simulink library "Hydraulic_Actuator_Lib"  (R2025a)
settings: Solver=ode45  StartTime=0.0  StopTime=10.0  RelTol=1e-3  EnableMultiTasking=on
undefined symbols (not defined in the file or in its folder): WT_Params
libraries: fl_lib x26, nesl_utility x9, SimscapeFluids_lib x7
Description:
  | Copyright 2009-2025 The MathWorks, Inc. MathWorks, Inc.
settings Model: Creator=smiller  LastModifiedBy=smiller
settings SolverCC: AlgebraicLoopSolver=TrustRegion
settings DataIOCC: LimitDataPoints=on  SaveFormat=Array  SignalLoggingSaveFormat=ModelDataLogs  ReturnWorkspaceOutputs=off
settings OptimizationCC: ReuseModelBlockBuffer=off  ExpressionDepthLimit=2147483647.0  LifeSpan=inf
settings DebuggingCC: UnderspecifiedInitializationDetection=Classic  MergeDetectMultiDrivingBlocksExec=none  SolverPrmCheckMsg=warning  FcnCallInpInsideContextMsg=warning  UnconnectedInputMsg=warning  UnconnectedOutputMsg=warning  UnconnectedLineMsg=warning  AllowSymbolicDim=off  StateNameClashWarn=warning  PregeneratedLibrarySubsystemCodeDiagnostic=none  SFUnexpectedBacktrackingDiag=warning  SFNoUnconditionalDefaultTransitionDiag=warning  SFExecutionAtInitializationDiag=none  ArithmeticOperatorsInVariantConditions=warning
settings HardwareCC: ProdBitPerPointer=32.0  ProdBitPerSizeT=32.0  ProdBitPerPtrDiffT=32.0  ProdLargestAtomicFloat=None  ProdIntDivRoundTo=Undefined  ProdEndianess=Unspecified  ProdWordSize=32.0  ProdHWDeviceType=32-bit Generic
settings ModelReferenceCC: EnableRefExpFcnMdlSchedulingChecks=on  PropagateSignalLabelsOutOfModel=off
settings SFSimCC: SimUseLocalCustomCode=off  CustomCodeUndefinedFunction=UseInterfaceOnly
settings RTWCC: RTWUseLocalCustomCode=off  GPUComputeCapability=3.5  DLArmComputeVersion=19.05
settings CodeAppCC: StateflowObjectComments=on
settings GRTTargetCC: TargetLangStandard=C89/C90 (ANSI)  CombineOutputUpdateFcns=off  GRTInterface=on
settings ConfigComp: CovMetricSettings=dw  CovSaveCumulativeToWorkspaceVar=on  CovSaveSingleToWorkspaceVar=on  CovExternalEMLEnable=off  CovSFcnEnable=off

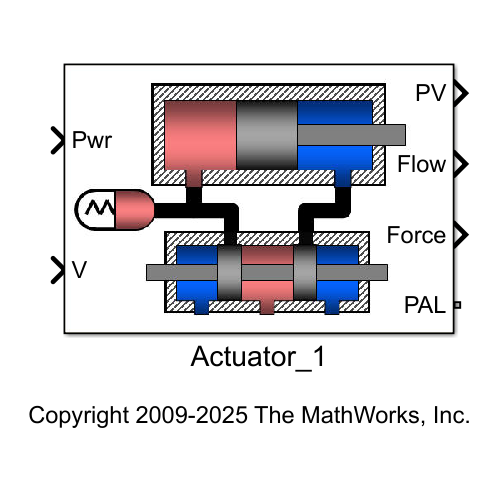
[thumbnail: Simulink's stored preview of the top-level diagram]
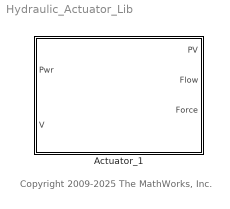
== system Hydraulic_Actuator_Lib ==
  note: Copyright 2009-2025 The MathWorks, Inc.
  Actuator_1 : Subsystem
      mask Display: image('Pitch_Hydraulic_Actuator_IMAGE.jpg');

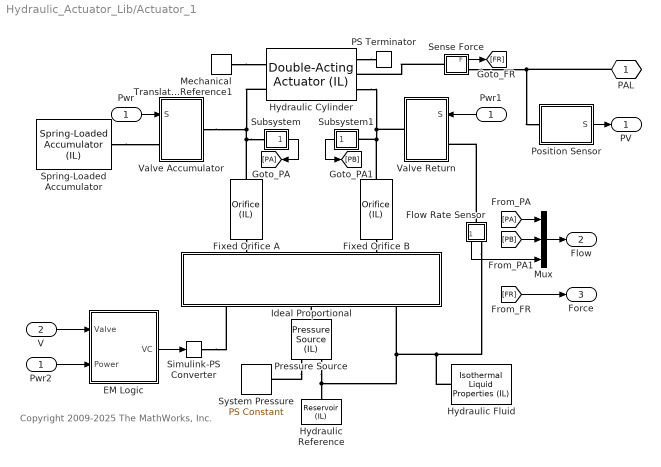
== system Hydraulic_Actuator_Lib/Actuator_1 ==
  note: Copyright 2009-2025 The MathWorks, Inc.
  Pwr : Inport
  V : Inport  Port=2
  EM Logic : Subsystem
  Fixed Orifice A : SimscapeFluids_lib/Isothermal Liquid/Valves & Orifices/Orifices/Orifice (IL)  orifice_type=1  constant_orifice_spec=fluids.isothermal_liquid.valves_orifices.orifices.enum.constant_orifice_spec.area  variable_orifice_spec=fluids.isothermal_liquid.valves_orifices.orifices.enum.orifice_spec.linear  orifice_area_constant=WT_Params.Pitch_Actuator.orifice_area m^2  p_diff_TLU_constant=[-4, -3, -2, -1, -.5, 0, .5, 1, 2, 3, 4] MPa  vol_flow_TLU_constant=[-2.44, -2.12, -1.68, -1.22, -.84, 0, .85, 1.21, 1.7, 2.09, 2.41] .* 1e-3 m^3/s  S_min=0 m  del_S=5e-3 m  open_orientation=fluids.isothermal_liquid.valves_orifices.orifices.enum.orifice_orientation.positive  area_max=1e-4 m^2  area_leak=1e-10 m^2  S_TLU=[0, .002, .004, .007, .017] m  orifice_area_TLU=[1e-09, 2.0352e-07, 4.0736e-05, .00011438, .00034356] m^2  area=inf m^2  Cd=0.7  Re_c=12  smoothing_factor=0.01  pressure_recovery=false  S_vol_flow_TLU=[0, .002, .004, .007, .017] m  p_diff_TLU=[.3, .5, .7] MPa  vol_flow_TLU=1e-3 * [1.7e-05, 2e-05, 2.6e-05; .0035, .0045, .0053; .7, .9, 1.06; 1.96, 2.5, 3; 6, 7.7, 9.13] m^3/s
      settings: LibrarySourceBlock=sh_lib/Orifices/Fixed Orifice  InternalSimscapePortConfiguration="{\"Bottom\":[],\"Left\":[{\"id\":\"A\",\"label\":\"A\",\"type\":\"foundation.isothermal_liquid.isothermal_liquid\"}],\"Right\":[{\"id\":\"B\",\"label\":\"B\",\"type\":\"foundation.isothermal_liquid.isothermal_liquid\"}],\"Top\":[]}"
  Fixed Orifice B : SimscapeFluids_lib/Isothermal Liquid/Valves & Orifices/Orifices/Orifice (IL)  orifice_type=1  constant_orifice_spec=fluids.isothermal_liquid.valves_orifices.orifices.enum.constant_orifice_spec.area  variable_orifice_spec=fluids.isothermal_liquid.valves_orifices.orifices.enum.orifice_spec.linear  orifice_area_constant=WT_Params.Pitch_Actuator.orifice_area m^2  p_diff_TLU_constant=[-4, -3, -2, -1, -.5, 0, .5, 1, 2, 3, 4] MPa  vol_flow_TLU_constant=[-2.44, -2.12, -1.68, -1.22, -.84, 0, .85, 1.21, 1.7, 2.09, 2.41] .* 1e-3 m^3/s  S_min=0 m  del_S=5e-3 m  open_orientation=fluids.isothermal_liquid.valves_orifices.orifices.enum.orifice_orientation.positive  area_max=1e-4 m^2  area_leak=1e-10 m^2  S_TLU=[0, .002, .004, .007, .017] m  orifice_area_TLU=[1e-09, 2.0352e-07, 4.0736e-05, .00011438, .00034356] m^2  area=inf m^2  Cd=0.7  Re_c=12  smoothing_factor=0.01  pressure_recovery=false  S_vol_flow_TLU=[0, .002, .004, .007, .017] m  p_diff_TLU=[.3, .5, .7] MPa  vol_flow_TLU=1e-3 * [1.7e-05, 2e-05, 2.6e-05; .0035, .0045, .0053; .7, .9, 1.06; 1.96, 2.5, 3; 6, 7.7, 9.13] m^3/s
      settings: LibrarySourceBlock=sh_lib/Orifices/Fixed Orifice  InternalSimscapePortConfiguration="{\"Bottom\":[],\"Left\":[{\"id\":\"A\",\"label\":\"A\",\"type\":\"foundation.isothermal_liquid.isothermal_liquid\"}],\"Right\":[{\"id\":\"B\",\"label\":\"B\",\"type\":\"foundation.isothermal_liquid.isothermal_liquid\"}],\"Top\":[]}"
  Flow Rate Sensor : Subsystem
      mask Display: disp('F')
  Hydraulic Reference : fl_lib/Isothermal Liquid/Elements/Reservoir (IL)  reservoir_type=foundation.enum.constant_controlled.constant  pressure_spec=foundation.enum.pressure_spec.atmospheric  reservoir_pressure=0.101325 MPa
      settings: LibrarySourceBlock=fl_lib/Hydraulic/Hydraulic Elements/Hydraulic Reference
  Hydraulic Cylinder : SimscapeFluids_lib/Isothermal Liquid/Actuators/Double-Acting Actuator (IL)  single_fluid=true  mech_orientation=-1  piston_area_A=WT_Params.Pitch_Actuator.Cylinder.piston_area m^2  piston_area_B=WT_Params.Pitch_Actuator.Cylinder.piston_area m^2  stroke=WT_Params.Pitch_Actuator.Cylinder.stroke m  dead_volume_A=1e-04 m^3  dead_volume_B=1e-04 m^3  pressure_spec=foundation.enum.pressure_spec.atmospheric  environment_pressure=0.101325 MPa  hardstop_model=3  stiff_coeff=WT_Params.Pitch_Actuator.Cylinder.contact_stiffness N/m  damping_coeff=WT_Params.Pitch_Actuator.Cylinder.contact_damping N/(m/s)  transition=0.1 mm  coeff_rest=0.7  v_tol=0.001 m/s  f_tol=0.001 N  cushion_A_spec=false  area_plunger_A=1e-4 m^2  length_plunger_A=1e-3 m  area_cushion_orifice_A=1e-6 m^2  area_leak_plunger_A=1e-7 m^2  p_crack_differential_A=0.01 MPa  press_max_differential_A=0.1 MPa  check_valve_area_max_A=1e-4 m^2  check_valve_area_leak_A=1e-10 m^2  smoothing_factor_A=0  cushion_B_spec=false  area_plunger_B=1e-4 m^2  length_plunger_B=1e-3 m  area_cushion_orifice_B=1e-6 m^2  area_leak_plunger_B=1e-7 m^2  p_crack_differential_B=0.01 MPa  press_max_differential_B=0.1 MPa  check_valve_area_max_B=1e-4 m^2  check_valve_area_leak_B=1e-10 m^2  smoothing_factor_B=0  friction_spec=false  breakaway_Coulomb_ratio=1.2  breakaway_velocity=0.1 m/s  preload_force=20 N  Coulomb_coeff=1e-6 N/Pa  viscous_coeff=100 N*s/m  leakage_spec=false  clearance=1e-4 m  piston_length=0.01 m  displacement_spec=foundation.enum.DisplacementSpec.Calculate  x0=-(WT_Params.Pitch_Actuator.Cylinder.initial_disp_from_a) m  dynamic_compressibility=true  p0_A=0 + 101325 Pa  p0_B=0 + 101325 Pa  p_nominal_A=0.101325 MPa  p_nominal_B=0.101325 MPa
      settings: InternalSimscapePortConfiguration="{\"Bottom\":[],\"Left\":[{\"id\":\"C\",\"label\":\"C\",\"type\":\"foundation.mechanical.translational.translational\"},{\"id\":\"A\",\"label\":\"A\",\"type\":\"foundation.isothermal_liquid.isothermal_liquid\"}],\"Right\":[{\"id\":\"p_out\",\"label\":\"p\",\"type\":\"output\"},{\"id\":\"R\",\"label\":\"R\",\"type\":\"foundation.mechanical.translational.translational\"},{\"id\":\"B\",\"label\":\"B\",\"type\":\"foundation.isothermal_liquid.isothermal_liquid\"}],\"Top\":[]}"
      settings: LibrarySourceBlock=|
      | sh_lib/Hydraulic Cylinders/Double-Acting
      | Hydraulic Cylinder
  Hydraulic Fluid : fl_lib/Isothermal Liquid/Utilities/Isothermal Liquid Properties (IL)  rho_L_atm=961.8732 kg/m^3  bulk_modulus_model=foundation.enum.bulk_modulus_model.const  beta_gain=6  beta_L_atm=1.24285e+09 Pa  nu_atm=(7.1283)*(1) cSt  p_atm=0.101325 MPa  p_min=1 Pa  properties_range_check=simscape.enum.assert.action.error  air_fraction=0.005  polytropic_index=1.0  rho_g_atm=1.225 kg/m^3  air_dissolution_model=simscape.enum.onoff.off  p_crit=3 MPa
      settings: LibrarySourceBlock=sh_lib/Hydraulic Utilities/Hydraulic Fluid
  Ideal Proportional : Subsystem
      mask Display:
      | plot([198.418507352471;198.418507352471], [5.66910021007061;25.5109509453177])
      | plot([189.914857037365;206.922157667577], [25.5109509453177;25.5109509453177])
      | plot([240.936758928001;240.936758928001], [5.66910021007061;25.5109509453177])
      | plot([232.433108612895;249.440409243107], [25.5109509453177;25.5109509453177])
      | plot([240.936758928001;240.936758928001], [76.5328528359532;56.6910021007061])
      | plot([232.433108612895;249.440409243107], [56.6910021007061;56.6910021007061])
      | plot([198.418507352471;198.418507352471], [76.5328528359532;56.6910021007061])
      | plot([189.914857037365;206.922157667577], [56.6910021007061;56.6910021007061])
      | plot([99.2092536762357;99.2092536762357], [76.5328528359532;5.66910021007061])
      | plot([141.727505251765;141.727505251765], [76.5328528359532;5.66910021007061])
      | plot([170.073006302118;170.073006302118], [76.5328528359532;5.66910021007061])
      | plot([269.282259978354;269.282259978354], [76.5328528359532;5.66910021007061])
      | patch([99.2092536762357;93.5401534661651;104.878353886306;99.2092536762357], [76.5328528359532;53.8564519956708;53.8564519956708;76.5328528359532],[0 0 0])
      | plot([99.2092536762357;93.5401534661651;104.878353886306;99.2092536762357], [76.5328528359532;53.8564519956708;53.8564519956708;76.5328528359532])
      | patch([141.727505251765;136.058405041695;147.396605461836;141.727505251765], [5.66910021007061;28.3455010503531;28.3455010503531;5.66910021007061],[0 0 0])
      | plot([141.727505251765;136.058405041695;147.396605461836;141.727505251765], [5.66910021007061;28.3455010503531;28.3455010503531;5.66910021007061])
      | plot([297.627761028707;340.146012604237], [5.66910021007061;76.5328528359532])
      | plot([297.627761028707;340.146012604237], [76.5328528359532;5.66910021007061])
      | plot([70.8637526258826;368.49151365459;368.49151365459;70.8637526258826;70.8637526258826], [76.5328528359532;76.5328528359532;5.66910021007061;5.66910021007061;76.5328528359532])
      | patch([297.627761028707;303.296861238778;311.800511553884;297.627761028707], [5.66910021007061;25.5109509453177;19.8418507352471;5.66910021007061],[0 0 0])
      | plot([297.627761028707;303.296861238778;311.800511553884;297.627761028707], [5.66910021007061;25.5109509453177;19.8418507352471;5.66910021007061])
      | patch([297.627761028707;303.296861238778;311.800511553884;297.627761028707], [76.5328528359532;56.6910021007061;62.3601023107767;76.5328528359532],[0 0 0])
      | plot([297.627761028707;303.296861238778;311.800511553884;297.627761028707], [76.5328528359532;56.6910021007061;62.3601023107767;76.5328528359532])
      | plot([62.3601023107767;374.16061386466], [82.2019530460238;82.2019530460238])
      | plot([65.194652415812;376.995163969696], [0;0])
      | plot([70.8637526258826;0;0;70.8637526258826;70.8637526258826], [53.8564519956708;53.8564519956708;25.5109509453177;25.5109509453177;53.8564519956708]-25.5109509453177+5.66910021007061)
      | plot([70.8637526258826;0;0;70.8637526258826;70.8637526258826]+368.49151365459, [53.8564519956708;53.8564519956708;25.5109509453177;25.5109509453177;53.8564519956708]-25.5109509453177+5.66910021007061)
      | plot([15 25], [5.66910021007061 35])
      | plot([25 15]+405, [5.66910021007061 35])
      | plot([42.5 40]+5,[70 58]);
      | plot([45 50]+2.5,[70 45]);
      | plot([45 50]+7.5,[45 70]);
      | plot([45 50]+12.5,[70 45]);
      | plot([45 50]+17.5,[45 70]);
      | plot([40 42.5]+27.5,[70 58]);
      | plot([42.5 40]+5+324,[70 58]);
      | plot([45 50]+2.5+324,[70 45]);
      | plot([45 50]+7.5+324,[45 70]);
      | plot([45 50]+12.5+324,[70 45]);
      | plot([45 50]+17.5+324,[45 70]);
      | plot([40 42.5]+27.5+324,[70 58]);
      | ;color('red');
      | port_label('LConn', 1,'A')
      | port_label('LConn', 2,'B')
      | port_label('RConn', 1,'S')
      | port_label('RConn', 2,'P')
      | port_label('RConn', 3,'T')
  Mechanical Translational Reference1 : fl_lib/Mechanical/Translational Elements/Mechanical Translational Reference  Tag=Factory Generic
  Mux : Mux  Inputs=3
  PS Terminator : fl_lib/Physical Signals/Sinks/PS Terminator
  Position Sensor : Subsystem
      mask Display:
      | plot([25.5109509453177;56.6910021007061;70.8637526258826;96.3747035712004;127.554754726589;155.900255776942;184.245756827295;212.591257877648;235.26765871793;252.274959348142;283.455010503531], [155.900255776942;155.900255776942;110.547454096377;198.418507352471;113.382004201412;198.418507352471;116.216554306448;198.418507352471;113.382004201412;155.900255776942;155.900255776942])
      | plot([155.900255776942;155.900255776942], [266.447709873319;198.418507352471])
      | patch([155.900255776942;170.073006302118;141.727505251765;155.900255776942], [198.418507352471;226.764008402824;226.764008402824;198.418507352471], [0;0;0])
      | plot([155.900255776942;170.073006302118;141.727505251765;155.900255776942], [198.418507352471;226.764008402824;226.764008402824;198.418507352471])
      | ;
      | color('red');
      | port_label('LConn', 1,'R')
      | port_label('output', 1,'P')
  Pressure Source : fl_lib/Isothermal Liquid/Sources/Pressure Source (IL)  source_type=foundation.enum.constant_controlled.controlled  pressure_differential=0 MPa
      settings: InternalSimscapePortConfiguration="{\"Bottom\":[],\"Left\":[{\"id\":\"A\",\"label\":\"A\",\"type\":\"foundation.isothermal_liquid.isothermal_liquid\"},{\"id\":\"P\",\"label\":\"P\",\"type\":\"input\"}],\"Right\":[{\"id\":\"B\",\"label\":\"B\",\"type\":\"foundation.isothermal_liquid.isothermal_liquid\"}],\"Top\":[]}"
      settings: LibrarySourceBlock=|
      | fl_lib/Hydraulic/Hydraulic Sources/Hydraulic Pressure
      | Source
  Pwr1 : InportShadow
  Pwr2 : InportShadow
  Sense Force : Subsystem
      mask Display: disp('F');
  Simulink-PS Converter : nesl_utility/Simulink-PS Converter  PhysicalDomain=network_engine_domain  SubClassName=ps_input  LeftPortType=input  RightPortType=output  PseudoPeriodic=off  Frequencies=[]  NoiseDistribution=none  NoiseParameters=[]  Unit=1  AffineConversion=off  FilteringAndDerivatives=zero  SimscapeFilterOrder=1  InputFilterTimeConstant=0.005  UdotUserProvided=0
  Spring-Loaded Accumulator : SimscapeFluids_lib/Isothermal Liquid/Tanks & Accumulators/Spring-Loaded Accumulator (IL)  capacity=WT_Params.Pitch_Actuator.Accumulator.capacity m^3  p_preload=WT_Params.Pitch_Actuator.Accumulator.preload_pressure + 101325 Pa  p_max=WT_Params.Pitch_Actuator.Accumulator.maximum_pressure + 101325 Pa  stiff_coeff=1e4 Pa/m^3  dynamic_compressibility=simscape.enum.onoff.off  liquid_volume_specify=on  liquid_volume_priority=High  liquid_volume=WT_Params.Pitch_Actuator.Accumulator.initial_volume m^3  liquid_volume_nominal_specify=off  liquid_volume_nominal_value=1  liquid_volume_nominal_unit=m^3  liquid_mass_specify=off  liquid_mass_priority=None  liquid_mass=5 kg  liquid_mass_nominal_specify=off  liquid_mass_nominal_value=1  liquid_mass_nominal_unit=kg  p_I_specify=on  p_I_priority=None  p_I=1.01325e5 + 101325 Pa  p_I_nominal_specify=off  p_I_nominal_value=1  p_I_nominal_unit=Pa
      settings: InternalSimscapePortConfiguration="{\"Bottom\":[],\"Left\":[],\"Right\":[{\"id\":\"A\",\"label\":\"A\",\"type\":\"foundation.isothermal_liquid.isothermal_liquid\"}],\"Top\":[]}"
      settings: LibrarySourceBlock=|
      | sh_lib/Accumulators/Spring-Loaded
      | Accumulator
  Subsystem : Subsystem
      mask Display: disp('P')
  Subsystem1 : Subsystem
      mask Display: disp('P')
  System Pressure : fl_lib/Physical Signals/Sources/PS Constant  constant=WT_Params.Pitch_Actuator.hydraulic_pressure
  Valve Accumulator : Subsystem
      mask Display:
      | plot([73.6983027309179;124.720204621553], [181.41120672226;181.41120672226])
      | plot([76.2808928266168;277.78591029346], [385.498814284801;385.498814284801])
      | plot([77.0997628569603;276.967040263116], [283.455010503531;283.455010503531])
      | plot([73.6983027309179;276.967040263116;276.967040263116;73.6983027309179;73.6983027309179], [487.542618066072;487.542618066072;79.3674029409885;79.3674029409885;487.542618066072])
      | plot([277.78591029346;226.764008402824], [181.41120672226;181.285226717591])
      | plot([226.764008402824;226.764008402824], [205.28441760689;157.286035828292])
      | patch([206.35524764657;206.35524764657;280.368500389159;206.35524764657], [400.805384851992;370.192243717611;385.498814284801;400.805384851992], [0;0;0])
      | plot([206.35524764657;206.35524764657;280.368500389159;206.35524764657], [400.805384851992;370.192243717611;385.498814284801;400.805384851992])
      | plot([124.720204621553;124.720204621553], [204.906477592885;156.971085816622])
      | plot([0;351.484213024378;351.484213024378;0;0], [566.910021007061;566.910021007061;0;0;566.910021007061])
      | ;
      | color('red');
      | port_label('input', 1,'S');
      | port_label('lconn', 1,'A');
      | port_label('rconn', 1,'B');
  Valve Return : Subsystem
      mask Display:
      | plot([73.6983027309179;124.720204621553], [181.41120672226;181.41120672226])
      | plot([76.2808928266168;277.78591029346], [385.498814284801;385.498814284801])
      | plot([77.0997628569603;276.967040263116], [283.455010503531;283.455010503531])
      | plot([73.6983027309179;276.967040263116;276.967040263116;73.6983027309179;73.6983027309179], [487.542618066072;487.542618066072;79.3674029409885;79.3674029409885;487.542618066072])
      | plot([277.78591029346;226.764008402824], [181.41120672226;181.285226717591])
      | plot([226.764008402824;226.764008402824], [205.28441760689;157.286035828292])
      | patch([206.35524764657;206.35524764657;280.368500389159;206.35524764657], [400.805384851992;370.192243717611;385.498814284801;400.805384851992], [0;0;0])
      | plot([206.35524764657;206.35524764657;280.368500389159;206.35524764657], [400.805384851992;370.192243717611;385.498814284801;400.805384851992])
      | plot([124.720204621553;124.720204621553], [204.906477592885;156.971085816622])
      | plot([0;351.484213024378;351.484213024378;0;0], [566.910021007061;566.910021007061;0;0;566.910021007061])
      | ;
      | color('red');
      | port_label('input', 1,'S');
      | port_label('lconn', 1,'A');
      | port_label('rconn', 1,'B');
  PAL : PMIOPort  Tag=PMCPort  Side=Right
  PV : Outport  VectorParamsAs1DForOutWhenUnconnected=off
  Flow : Outport  Port=2  VectorParamsAs1DForOutWhenUnconnected=off
  Force : Outport  Port=3  VectorParamsAs1DForOutWhenUnconnected=off
  wires:
  Pwr2/1 -> EM Logic/2(Power)
  EM Logic/1(VC) -> Simulink-PS Converter/1
  [PB] -> Mux/2
  [PA] -> Mux/1
  Flow Rate Sensor/1(Flow) -> Mux/3
  Subsystem1/1(P) -> [PB]
  Subsystem/1(P) -> [PA]
  V/1 -> EM Logic/1(Valve)
  Pwr1/1 -> Valve Return/1(S)
  Pwr/1 -> Valve Accumulator/1(S)
  Position Sensor/1(S) -> PV/1
  Mux/1 -> Flow/1
  Sense Force/1(F) -> [FR]
  [FR] -> Force/1
  connections:
  Flow Rate Sensor/LConn1 -- Valve Return/LConn1
  Sense Force/RConn1 -- PAL/RConn1 -- Position Sensor/LConn1
  Spring-Loaded Accumulator/RConn1 -- Valve Accumulator/LConn1
  Ideal Proportional/RConn3 -- Pressure Source/LConn1 -- Hydraulic Reference/LConn1 -- Hydraulic Fluid/RConn1 -- Flow Rate Sensor/RConn1
  Simulink-PS Converter/RConn1 -- Ideal Proportional/RConn1
  Fixed Orifice A/LConn1 -- Ideal Proportional/LConn1
  Fixed Orifice B/LConn1 -- Ideal Proportional/LConn2
  Subsystem/LConn1 -- Fixed Orifice A/RConn1 -- Hydraulic Cylinder/LConn2 -- Valve Accumulator/RConn1
  Subsystem1/LConn1 -- Fixed Orifice B/RConn1 -- Hydraulic Cylinder/RConn3 -- Valve Return/RConn1
  Mechanical Translational Reference1/LConn1 -- Hydraulic Cylinder/LConn1
  Sense Force/LConn1 -- Hydraulic Cylinder/RConn2
  Pressure Source/RConn1 -- Ideal Proportional/RConn2
  Pressure Source/LConn2 -- System Pressure/RConn1
  Hydraulic Cylinder/RConn1 -- PS Terminator/LConn1

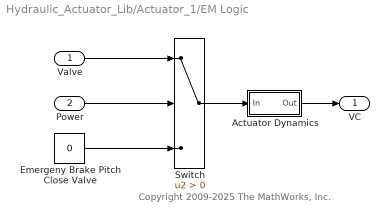
== system Hydraulic_Actuator_Lib/Actuator_1/EM Logic ==
  note: Copyright 2009-2025 The MathWorks, Inc.
  Valve : Inport
  Power : Inport  Port=2
  Actuator Dynamics : Subsystem  mask(First-order lag supporting vector signals){b=WT_Params.Pitch_Actuator.hydraulic_actuator_time_constant, x_initial=0}
      mask prompts: b "Filter time constant"; x_initial "Initial output"
      mask help: Models a lag of the form 1/(b*s+1) where s is the Laplace operator.
  Emergeny Brake Pitch Close Valve : Constant  Value=0
  Switch : Switch  Criteria=u2 > Threshold  SaturateOnIntegerOverflow=off  InputSameDT=off
  VC : Outport  VectorParamsAs1DForOutWhenUnconnected=off
  wires:
  Switch/1 -> Actuator Dynamics/1(In)
  Emergeny Brake Pitch Close Valve/1 -> Switch/3
  Power/1 -> Switch/2
  Valve/1 -> Switch/1
  Actuator Dynamics/1(Out) -> VC/1

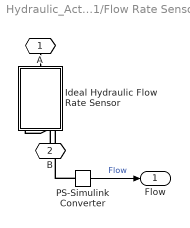
== system Hydraulic_Actuator_Lib/Actuator_1/Flow Rate Sensor ==
  Ideal Hydraulic Flow Rate Sensor : Subsystem
  PS-Simulink Converter : nesl_utility/PS-Simulink Converter  PhysicalDomain=network_engine_domain  SubClassName=ps_output  LeftPortType=input  RightPortType=output  PseudoPeriodic=off  Frequencies=[]  VectorFormat=1-D array  Unit=1  AffineConversion=off
  A : PMIOPort  Side=Left
  B : PMIOPort  Port=2  Side=Right
  Flow : Outport  VectorParamsAs1DForOutWhenUnconnected=off
  wires:
  PS-Simulink Converter/1 -> Flow/1  "Flow"
  connections:
  A/RConn1 -- Ideal Hydraulic Flow Rate Sensor/LConn1
  B/RConn1 -- Ideal Hydraulic Flow Rate Sensor/RConn1
  PS-Simulink Converter/LConn1 -- Ideal Hydraulic Flow Rate Sensor/RConn3

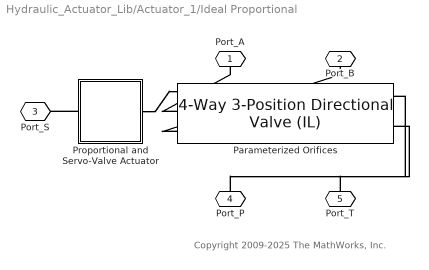
== system Hydraulic_Actuator_Lib/Actuator_1/Ideal Proportional ==
  note: Copyright 2009-2025 The MathWorks, Inc.
  Parameterized Orifices : SimscapeFluids_lib/Isothermal Liquid/Valves & Orifices/Directional Control Valves/4-Way 3-Position Directional Valve (IL)  open_orifices_pos=fluids.isothermal_liquid.valves_orifices.directional_control_valves.enum.directional_valve_open_orifices_pos_neg.PA_BT  open_orifices_neu=fluids.isothermal_liquid.valves_orifices.directional_control_valves.enum.directional_valve_open_orifices_neutral.all_closed  open_orifices_neg=fluids.isothermal_liquid.valves_orifices.directional_control_valves.enum.directional_valve_open_orifices_pos_neg.PB_AT  neutral_assert_action=0  area_spec=1  valve_spec=1  del_S_max=(WT_Params.Pitch_Actuator.Valve.max_opening) - (WT_Params.Pitch_Actuator.Valve.max_opening)/(WT_Params.Pitch_Actuator.Valve.max_area)*(WT_Params.Pitch_Actuator.Valve.leakage_area) m  area_max=WT_Params.Pitch_Actuator.Valve.max_area m^2  del_S_TLU=[0, .00125, .0025, .00375, .005] m  valve_area_TLU="[  1e-09 2.0352e-07 4.0736e-05 0.00011438 0.00034356 ] m^2"  del_S_vol_flow_TLU=[0, .00125, .0025, .00375, .005] m  p_diff_TLU="[  -1e+07 -5e+06 -2e+06 2e+06 5e+06 1e+07 ] Pa"  vol_flow_TLU="[  -1e-07 -7.0711e-08 -4.4721e-08 4.4721e-08 7.0711e-08 1e-07 ; -2.0352e-05 -1.4391e-05 -9.1017e-06 9.1017e-06 1.4391e-05 2.0352e-05 ; -0.0040736 -0.0028805 -0.0018218 0.0018218 0.0028805 0.0040736 ; -0.011438 -0.0080879 -0.0051152 0.0051152 0.0080879 0.011438 ; -0.034356 -0.024293 -0.015364 0.015364 0.024293 0.034356 ; ] m^3/s"  p_diff_TLU_const=[-.1, .3, .5, .7] MPa  vol_flow_TLU_const=[-.0009, .0016, .002, .0024] m^3/s  area_const=1e-4 m^2  area_leak=WT_Params.Pitch_Actuator.Valve.leakage_area m^2  area=inf m^2  Cd=0.7  Re_c=12  smoothing_factor=0  pressure_recovery=false  S_max_PA=-(WT_Params.Pitch_Actuator.Valve.initial_opening_pa) + (WT_Params.Pitch_Actuator.Valve.max_opening) m  del_S_max_PA=(0.005) - (0.005)/(0.5e-4)*(WT_Params.Pitch_Actuator.Valve.leakage_area) m  area_max_PA=0.5e-4 m^2  del_S_TLU_PA=[0, .00125, .0025, .00375, .005] m  valve_area_TLU_PA=[1.0e-9, 2.0352e-7, 4.0736e-5, 0.00011438, 0.00034356] m^2  del_S_vol_flow_TLU_PA=[0, .00125, .0025, .00375, .005] m  p_diff_TLU_PA=[-10000000.0, -5000000.0, -2000000.0, 2000000.0, 5000000.0, 10000000.0] Pa  vol_flow_TLU_PA=[-1.0e-7, -7.0711e-8, -4.4721e-8, 4.4721e-8, 7.0711e-8, 1.0e-7; -2.0352e-5, -1.4391e-5, -9.1017e-6, 9.1017e-6, 1.4391e-5, 2.0352e-5; -0.0040736, -0.0028805, -0.0018218, 0.0018218, 0.0028805, 0.0040736; -0.011438, -0.0080879, -0.0051152, 0.0051152, 0.0080879, 0.011438; -0.034356, -0.024293, -0.015364, 0.015364, 0.024293, 0.034356] m^3/s  area_const_PA=1e-4 m^2  p_diff_TLU_const_PA=[-.1, .3, .5, .7] MPa  vol_flow_TLU_const_PA=[-.0009, .0016, .002, .0024] m^3/s  S_max_PB=(WT_Params.Pitch_Actuator.Valve.initial_opening_pb) - (WT_Params.Pitch_Actuator.Valve.max_opening) m  del_S_max_PB=(0.005) - (0.005)/(0.5e-4)*(WT_Params.Pitch_Actuator.Valve.leakage_area) m  area_max_PB=0.5e-4 m^2  del_S_TLU_PB=[0, .00125, .0025, .00375, .005] m  valve_area_TLU_PB=[1.0e-9, 2.0352e-7, 4.0736e-5, 0.00011438, 0.00034356] m^2  del_S_vol_flow_TLU_PB=[0, .00125, .0025, .00375, .005] m  p_diff_TLU_PB=[-10000000.0, -5000000.0, -2000000.0, 2000000.0, 5000000.0, 10000000.0] Pa  vol_flow_TLU_PB=[-1.0e-7, -7.0711e-8, -4.4721e-8, 4.4721e-8, 7.0711e-8, 1.0e-7; -2.0352e-5, -1.4391e-5, -9.1017e-6, 9.1017e-6, 1.4391e-5, 2.0352e-5; -0.0040736, -0.0028805, -0.0018218, 0.0018218, 0.0028805, 0.0040736; -0.011438, -0.0080879, -0.0051152, 0.0051152, 0.0080879, 0.011438; -0.034356, -0.024293, -0.015364, 0.015364, 0.024293, 0.034356] m^3/s  area_const_PB=1e-4 m^2  p_diff_TLU_const_PB=[-.1, .3, .5, .7] MPa  vol_flow_TLU_const_PB=[-.0009, .0016, .002, .0024] m^3/s  S_max_AB=7.5e-3 m  del_S_max_AB=0.005 m  area_max_AB=1e-4 m^2  del_S_TLU_AB=[0, .00125, .0025, .00375, .005] m  valve_area_TLU_AB=[1e-10, 1e-05, 4e-05, 6e-05, .0001] m^2  del_S_vol_flow_TLU_AB=[0, .00125, .0025, .00375, .005] m  p_diff_TLU_AB=[-.1, .3, .5, .7] MPa  vol_flow_TLU_AB=[-1e-08, 2.2e-08, 2.8e-08, 3.4e-08; -9e-06, .00015, .0002, .00024; -.00036, .00063, .00081, .00096; -.00054, .00094, .0012, .0014; -.00091, .0016, .002, .0024] m^3/s  area_const_AB=1e-4 m^2  p_diff_TLU_const_AB=[-.1, .3, .5, .7] MPa  vol_flow_TLU_const_AB=[-.0009, .0016, .002, .0024] m^3/s  S_max_AT=(WT_Params.Pitch_Actuator.Valve.initial_opening_at) - (WT_Params.Pitch_Actuator.Valve.max_opening) m  del_S_max_AT=(0.005) - (0.005)/(0.5e-4)*(WT_Params.Pitch_Actuator.Valve.leakage_area) m  area_max_AT=0.5e-4 m^2  del_S_TLU_AT=[0, .00125, .0025, .00375, .005] m  valve_area_TLU_AT=[1.0e-9, 2.0352e-7, 4.0736e-5, 0.00011438, 0.00034356] m^2  del_S_vol_flow_TLU_AT=[0, .00125, .0025, .00375, .005] m  p_diff_TLU_AT=[-10000000.0, -5000000.0, -2000000.0, 2000000.0, 5000000.0, 10000000.0] Pa  vol_flow_TLU_AT=[-1.0e-7, -7.0711e-8, -4.4721e-8, 4.4721e-8, 7.0711e-8, 1.0e-7; -2.0352e-5, -1.4391e-5, -9.1017e-6, 9.1017e-6, 1.4391e-5, 2.0352e-5; -0.0040736, -0.0028805, -0.0018218, 0.0018218, 0.0028805, 0.0040736; -0.011438, -0.0080879, -0.0051152, 0.0051152, 0.0080879, 0.011438; -0.034356, -0.024293, -0.015364, 0.015364, 0.024293, 0.034356] m^3/s  area_const_AT=1e-4 m^2  p_diff_TLU_const_AT=[-.1, .3, .5, .7] MPa  vol_flow_TLU_const_AT=[-.0009, .0016, .002, .0024] m^3/s  S_max_BT=-(WT_Params.Pitch_Actuator.Valve.initial_opening_bt) + (WT_Params.Pitch_Actuator.Valve.max_opening) m  del_S_max_BT=(0.005) - (0.005)/(0.5e-4)*(WT_Params.Pitch_Actuator.Valve.leakage_area) m  area_max_BT=0.5e-4 m^2  del_S_TLU_BT=[0, .00125, .0025, .00375, .005] m  valve_area_TLU_BT=[1.0e-9, 2.0352e-7, 4.0736e-5, 0.00011438, 0.00034356] m^2  del_S_vol_flow_TLU_BT=[0, .00125, .0025, .00375, .005] m  p_diff_TLU_BT=[-10000000.0, -5000000.0, -2000000.0, 2000000.0, 5000000.0, 10000000.0] Pa  vol_flow_TLU_BT=[-1.0e-7, -7.0711e-8, -4.4721e-8, 4.4721e-8, 7.0711e-8, 1.0e-7; -2.0352e-5, -1.4391e-5, -9.1017e-6, 9.1017e-6, 1.4391e-5, 2.0352e-5; -0.0040736, -0.0028805, -0.0018218, 0.0018218, 0.0028805, 0.0040736; -0.011438, -0.0080879, -0.0051152, 0.0051152, 0.0080879, 0.011438; -0.034356, -0.024293, -0.015364, 0.015364, 0.024293, 0.034356] m^3/s  area_const_BT=1e-4 m^2  p_diff_TLU_const_BT=[-.1, .3, .5, .7] MPa  vol_flow_TLU_const_BT=[-.0009, .0016, .002, .0024] m^3/s  S_max_PT=0 m  del_S_max_PT=0.005 m  area_max_PT=1e-4 m^2  del_S_TLU_PT=[0, .00125, .0025, .00375, .005] m  valve_area_TLU_PT=[1e-10, 1e-05, 4e-05, 6e-05, .0001] m^2  del_S_vol_flow_TLU_PT=[0, .00125, .0025, .00375, .005] m  p_diff_TLU_PT=[-.1, .3, .5, .7] MPa  vol_flow_TLU_PT=[-1e-08, 2.2e-08, 2.8e-08, 3.4e-08; -9e-06, .00015, .0002, .00024; -.00036, .00063, .00081, .00096; -.00054, .00094, .0012, .0014; -.00091, .0016, .002, .0024] m^3/s
      settings: InternalSimscapePortConfiguration="{\"Bottom\":[{\"id\":\"P\",\"label\":\"P\",\"type\":\"foundation.isothermal_liquid.isothermal_liquid\"},{\"id\":\"T\",\"label\":\"T\",\"type\":\"foundation.isothermal_liquid.isothermal_liquid\"}],\"Left\":[{\"id\":\"S\",\"label\":\"S\",\"type\":\"input\"}],\"Right\":[],\"Top\":[{\"id\":\"A\",\"label\":\"A\",\"type\":\"foundation.isothermal_liquid.isothermal_liquid\"},{\"id\":\"B\",\"label\":\"B\",\"type\":\"foundation.isothermal_liquid.isothermal_liquid\"}]}"
      settings: LibrarySourceBlock=|
      | sh_lib/Valves/Directional Valves/4-Way Directional
      | Valve
  Proportional and Servo-Valve Actuator : Subsystem
  Port_A : PMIOPort  Side=Left
  Port_B : PMIOPort  Port=2  Side=Left
  Port_S : PMIOPort  Port=3  Side=Right
  Port_P : PMIOPort  Port=4  Side=Right
  Port_T : PMIOPort  Port=5  Side=Right
  connections:
  Parameterized Orifices/LConn2 -- Port_A/RConn1
  Parameterized Orifices/LConn3 -- Port_B/RConn1
  Port_P/RConn1 -- Parameterized Orifices/RConn1
  Proportional and Servo-Valve Actuator/LConn1 -- Port_S/RConn1
  Proportional and Servo-Valve Actuator/RConn1 -- Parameterized Orifices/LConn1
  Port_T/RConn1 -- Parameterized Orifices/RConn2

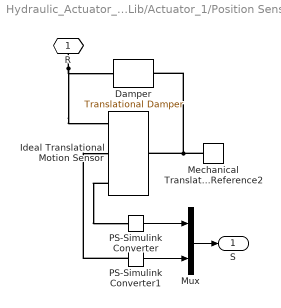
== system Hydraulic_Actuator_Lib/Actuator_1/Position Sensor ==
  Damper : fl_lib/Mechanical/Translational Elements/Translational Damper  D=WT_Params.Pitch_Actuator.Cylinder.damping N/(m/s)  v_specify=off  v_priority=High  v=0 m/s  v_nominal_specify=off  v_nominal_value=1  v_nominal_unit=m/s  f_specify=off  f_priority=High  f=0 N  f_nominal_specify=off  f_nominal_value=1  f_nominal_unit=N
  Ideal Translational Motion Sensor : fl_lib/Mechanical/Mechanical Sensors/Ideal Translational Motion Sensor  reference=foundation.enum.MeasurementReference.difference  acceleration_port=false  velocity_port=true  position_port=true  offset=WT_Params.Pitch_Actuator.Sensor.initial_position m
  Mechanical Translational Reference2 : fl_lib/Mechanical/Translational Elements/Mechanical Translational Reference  Tag=Factory Generic
  Mux : Mux  Inputs=2
  PS-Simulink Converter : nesl_utility/PS-Simulink Converter  PhysicalDomain=network_engine_domain  SubClassName=ps_output  LeftPortType=input  RightPortType=output  PseudoPeriodic=off  Frequencies=[]  VectorFormat=1-D array  Unit=1  AffineConversion=off
  PS-Simulink Converter1 : nesl_utility/PS-Simulink Converter  PhysicalDomain=network_engine_domain  SubClassName=ps_output  LeftPortType=input  RightPortType=output  PseudoPeriodic=off  Frequencies=[]  VectorFormat=1-D array  Unit=1  AffineConversion=off
  R : PMIOPort  Side=Left
  S : Outport  VectorParamsAs1DForOutWhenUnconnected=off
  wires:
  PS-Simulink Converter1/1 -> Mux/2
  Mux/1 -> S/1
  PS-Simulink Converter/1 -> Mux/1
  connections:
  PS-Simulink Converter1/LConn1 -- Ideal Translational Motion Sensor/RConn2
  Ideal Translational Motion Sensor/RConn3 -- PS-Simulink Converter/LConn1
  Mechanical Translational Reference2/LConn1 -- Ideal Translational Motion Sensor/LConn1 -- Damper/RConn1
  R/RConn1 -- Damper/LConn1 -- Ideal Translational Motion Sensor/RConn1

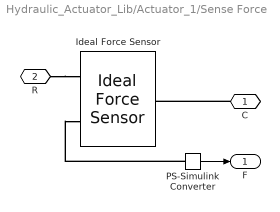
== system Hydraulic_Actuator_Lib/Actuator_1/Sense Force ==
  Ideal Force Sensor : fl_lib/Mechanical/Mechanical Sensors/Ideal Force Sensor
  PS-Simulink Converter : nesl_utility/PS-Simulink Converter  PhysicalDomain=network_engine_domain  SubClassName=ps_output  LeftPortType=input  RightPortType=output  PseudoPeriodic=off  Frequencies=[]  VectorFormat=1-D array  Unit=1  AffineConversion=off
  C : PMIOPort  Side=Right
  R : PMIOPort  Port=2  Side=Left
  F : Outport  VectorParamsAs1DForOutWhenUnconnected=off
  wires:
  PS-Simulink Converter/1 -> F/1
  connections:
  PS-Simulink Converter/LConn1 -- Ideal Force Sensor/RConn2
  C/RConn1 -- Ideal Force Sensor/LConn1
  R/RConn1 -- Ideal Force Sensor/RConn1

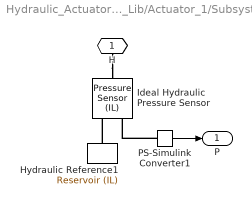
== system Hydraulic_Actuator_Lib/Actuator_1/Subsystem ==
  Hydraulic Reference1 : fl_lib/Isothermal Liquid/Elements/Reservoir (IL)  reservoir_type=foundation.enum.constant_controlled.constant  pressure_spec=foundation.enum.pressure_spec.atmospheric  reservoir_pressure=0.101325 MPa
      settings: LibrarySourceBlock=fl_lib/Hydraulic/Hydraulic Elements/Hydraulic Reference
  Ideal Hydraulic Pressure Sensor : fl_lib/Isothermal Liquid/Sensors/Pressure Sensor (IL)  pressure_measure=foundation.enum.pressure_measure.difference
      settings: InternalSimscapePortConfiguration="{\"Bottom\":[],\"Left\":[{\"id\":\"A\",\"label\":\"A\",\"type\":\"foundation.isothermal_liquid.isothermal_liquid\"}],\"Right\":[{\"id\":\"B\",\"label\":\"B\",\"type\":\"foundation.isothermal_liquid.isothermal_liquid\"},{\"id\":\"P\",\"label\":\"P\",\"type\":\"output\"}],\"Top\":[]}"
      settings: LibrarySourceBlock=|
      | fl_lib/Hydraulic/Hydraulic Sensors/Hydraulic Pressure
      | Sensor
  PS-Simulink Converter1 : nesl_utility/PS-Simulink Converter  PhysicalDomain=network_engine_domain  SubClassName=ps_output  LeftPortType=input  RightPortType=output  PseudoPeriodic=off  Frequencies=[]  VectorFormat=1-D array  Unit=1  AffineConversion=off
  H : PMIOPort  Side=Left
  P : Outport  VectorParamsAs1DForOutWhenUnconnected=off
  wires:
  PS-Simulink Converter1/1 -> P/1
  connections:
  H/RConn1 -- Ideal Hydraulic Pressure Sensor/LConn1
  PS-Simulink Converter1/LConn1 -- Ideal Hydraulic Pressure Sensor/RConn2
  Hydraulic Reference1/LConn1 -- Ideal Hydraulic Pressure Sensor/RConn1

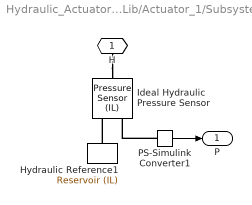
== system Hydraulic_Actuator_Lib/Actuator_1/Subsystem1 ==
  Hydraulic Reference1 : fl_lib/Isothermal Liquid/Elements/Reservoir (IL)  reservoir_type=foundation.enum.constant_controlled.constant  pressure_spec=foundation.enum.pressure_spec.atmospheric  reservoir_pressure=0.101325 MPa
      settings: LibrarySourceBlock=fl_lib/Hydraulic/Hydraulic Elements/Hydraulic Reference
  Ideal Hydraulic Pressure Sensor : fl_lib/Isothermal Liquid/Sensors/Pressure Sensor (IL)  pressure_measure=foundation.enum.pressure_measure.difference
      settings: InternalSimscapePortConfiguration="{\"Bottom\":[],\"Left\":[{\"id\":\"A\",\"label\":\"A\",\"type\":\"foundation.isothermal_liquid.isothermal_liquid\"}],\"Right\":[{\"id\":\"B\",\"label\":\"B\",\"type\":\"foundation.isothermal_liquid.isothermal_liquid\"},{\"id\":\"P\",\"label\":\"P\",\"type\":\"output\"}],\"Top\":[]}"
      settings: LibrarySourceBlock=|
      | fl_lib/Hydraulic/Hydraulic Sensors/Hydraulic Pressure
      | Sensor
  PS-Simulink Converter1 : nesl_utility/PS-Simulink Converter  PhysicalDomain=network_engine_domain  SubClassName=ps_output  LeftPortType=input  RightPortType=output  PseudoPeriodic=off  Frequencies=[]  VectorFormat=1-D array  Unit=1  AffineConversion=off
  H : PMIOPort  Side=Left
  P : Outport  VectorParamsAs1DForOutWhenUnconnected=off
  wires:
  PS-Simulink Converter1/1 -> P/1
  connections:
  Hydraulic Reference1/LConn1 -- Ideal Hydraulic Pressure Sensor/RConn1
  PS-Simulink Converter1/LConn1 -- Ideal Hydraulic Pressure Sensor/RConn2
  H/RConn1 -- Ideal Hydraulic Pressure Sensor/LConn1

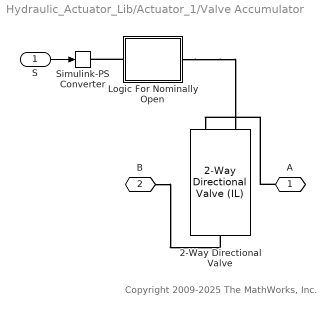
== system Hydraulic_Actuator_Lib/Actuator_1/Valve Accumulator ==
  note: Copyright 2009-2025 The MathWorks, Inc.
  S : Inport
  2-Way Directional Valve : SimscapeFluids_lib/Isothermal Liquid/Valves & Orifices/Directional Control Valves/2-Way Directional Valve (IL)  valve_spec=1  S_max=0.005 m  del_S_max=(0.005) - ((0.005)/(WT_Params.Pitch_Actuator.Emergency_Pitch_Valve.max_area)*(1e-12) - (0)) m  area_max=WT_Params.Pitch_Actuator.Emergency_Pitch_Valve.max_area m^2  area_leak=1e-12 m^2  del_S_TLU="[0       0.002       0.004       0.007       0.017] m"  orifice_area_TLU="[  1e-09 2.0352e-07 4.0736e-05 0.00011438 0.00034356 ] m^2"  del_S_vol_flow_TLU="[0       0.002       0.004       0.007       0.017] m"  p_diff_TLU="[  -1e+07 -5e+06 -2e+06 2e+06 5e+06 1e+07 ] Pa"  vol_flow_TLU="[  -1e-07 -7.0711e-08 -4.4721e-08 4.4721e-08 7.0711e-08 1e-07 ; -2.0352e-05 -1.4391e-05 -9.1017e-06 9.1017e-06 1.4391e-05 2.0352e-05 ; -0.0040736 -0.0028805 -0.0018218 0.0018218 0.0028805 0.0040736 ; -0.011438 -0.0080879 -0.0051152 0.0051152 0.0080879 0.011438 ; -0.034356 -0.024293 -0.015364 0.015364 0.024293 0.034356 ; ] m^3/s"  Cd=0.7  Re_c=12  smoothing_factor=0  pressure_recovery=false  area=inf m^2
      settings: InternalSimscapePortConfiguration="{\"Bottom\":[{\"id\":\"B\",\"label\":\"B\",\"type\":\"foundation.isothermal_liquid.isothermal_liquid\"}],\"Left\":[{\"id\":\"S\",\"label\":\"S\",\"type\":\"input\"}],\"Right\":[],\"Top\":[{\"id\":\"A\",\"label\":\"A\",\"type\":\"foundation.isothermal_liquid.isothermal_liquid\"}]}"
      settings: LibrarySourceBlock=|
      | sh_lib/Valves/Directional Valves/2-Way Directional
      | Valve
  Logic For Nominally Open : Subsystem
  Simulink-PS Converter : nesl_utility/Simulink-PS Converter  PhysicalDomain=network_engine_domain  SubClassName=ps_input  LeftPortType=input  RightPortType=output  PseudoPeriodic=off  Frequencies=[]  NoiseDistribution=none  NoiseParameters=[]  Unit=1  AffineConversion=off  FilteringAndDerivatives=zero  SimscapeFilterOrder=1  InputFilterTimeConstant=0.005  UdotUserProvided=0
  A : PMIOPort  Side=Left
  B : PMIOPort  Port=2  Side=Right
  wires:
  S/1 -> Simulink-PS Converter/1
  connections:
  Logic For Nominally Open/RConn1 -- 2-Way Directional Valve/LConn1
  B/RConn1 -- 2-Way Directional Valve/RConn1
  A/RConn1 -- 2-Way Directional Valve/LConn2
  Logic For Nominally Open/LConn1 -- Simulink-PS Converter/RConn1

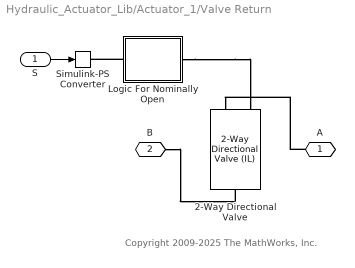
== system Hydraulic_Actuator_Lib/Actuator_1/Valve Return ==
  note: Copyright 2009-2025 The MathWorks, Inc.
  S : Inport
  2-Way Directional Valve : SimscapeFluids_lib/Isothermal Liquid/Valves & Orifices/Directional Control Valves/2-Way Directional Valve (IL)  valve_spec=1  S_max=0.005 m  del_S_max=(0.005) - ((0.005)/(WT_Params.Pitch_Actuator.Emergency_Pitch_Valve.max_area)*(1e-12) - (0)) m  area_max=WT_Params.Pitch_Actuator.Emergency_Pitch_Valve.max_area m^2  area_leak=1e-12 m^2  del_S_TLU="[0       0.002       0.004       0.007       0.017] m"  orifice_area_TLU="[  1e-09 2.0352e-07 4.0736e-05 0.00011438 0.00034356 ] m^2"  del_S_vol_flow_TLU="[0       0.002       0.004       0.007       0.017] m"  p_diff_TLU="[  -1e+07 -5e+06 -2e+06 2e+06 5e+06 1e+07 ] Pa"  vol_flow_TLU="[  -1e-07 -7.0711e-08 -4.4721e-08 4.4721e-08 7.0711e-08 1e-07 ; -2.0352e-05 -1.4391e-05 -9.1017e-06 9.1017e-06 1.4391e-05 2.0352e-05 ; -0.0040736 -0.0028805 -0.0018218 0.0018218 0.0028805 0.0040736 ; -0.011438 -0.0080879 -0.0051152 0.0051152 0.0080879 0.011438 ; -0.034356 -0.024293 -0.015364 0.015364 0.024293 0.034356 ; ] m^3/s"  Cd=0.7  Re_c=12  smoothing_factor=0  pressure_recovery=false  area=inf m^2
      settings: InternalSimscapePortConfiguration="{\"Bottom\":[{\"id\":\"B\",\"label\":\"B\",\"type\":\"foundation.isothermal_liquid.isothermal_liquid\"}],\"Left\":[{\"id\":\"S\",\"label\":\"S\",\"type\":\"input\"}],\"Right\":[],\"Top\":[{\"id\":\"A\",\"label\":\"A\",\"type\":\"foundation.isothermal_liquid.isothermal_liquid\"}]}"
      settings: LibrarySourceBlock=|
      | sh_lib/Valves/Directional Valves/2-Way Directional
      | Valve
  Logic For Nominally Open : Subsystem
  Simulink-PS Converter : nesl_utility/Simulink-PS Converter  PhysicalDomain=network_engine_domain  SubClassName=ps_input  LeftPortType=input  RightPortType=output  PseudoPeriodic=off  Frequencies=[]  NoiseDistribution=none  NoiseParameters=[]  Unit=1  AffineConversion=off  FilteringAndDerivatives=zero  SimscapeFilterOrder=1  InputFilterTimeConstant=0.005  UdotUserProvided=0
  A : PMIOPort  Side=Left
  B : PMIOPort  Port=2  Side=Right
  wires:
  S/1 -> Simulink-PS Converter/1
  connections:
  Logic For Nominally Open/LConn1 -- Simulink-PS Converter/RConn1
  A/RConn1 -- 2-Way Directional Valve/LConn2
  B/RConn1 -- 2-Way Directional Valve/RConn1
  Logic For Nominally Open/RConn1 -- 2-Way Directional Valve/LConn1

== system Hydraulic_Actuator_Lib/Actuator_1/EM Logic/Actuator Dynamics ==
  note: Copyright 2009-2025 The MathWorks, Inc.
  In : Inport
  Gain : Gain  Gain=1/b
  Integrator : Integrator  InitialCondition=x_initial
  Sum : Sum  Inputs=|+-  InputSameDT=on  SaturateOnIntegerOverflow=on  OutDataTypeStr=Inherit: Same as first input
  Out : Outport  VectorParamsAs1DForOutWhenUnconnected=off
  wires:
  Gain/1 -> Out/1, Sum/2
  Integrator/1 -> Gain/1
  In/1 -> Sum/1
  Sum/1 -> Integrator/1

== system Hydraulic_Actuator_Lib/Actuator_1/Flow Rate Sensor/Ideal Hydraulic Flow Rate Sensor ==
  Ideal Hydraulic Flow Rate Sensor : fl_lib/Isothermal Liquid/Sensors/Flow Rate Sensor (IL)  sensor_type=3
      settings: InternalSimscapePortConfiguration="{\"Bottom\":[],\"Left\":[{\"id\":\"A\",\"label\":\"A\",\"type\":\"foundation.isothermal_liquid.isothermal_liquid\"}],\"Right\":[{\"id\":\"B\",\"label\":\"B\",\"type\":\"foundation.isothermal_liquid.isothermal_liquid\"},{\"id\":\"M\",\"label\":\"M\",\"type\":\"output\"},{\"id\":\"V\",\"label\":\"V\",\"type\":\"output\"}],\"Top\":[]}"
      settings: LibrarySourceBlock=|
      | fl_lib/Hydraulic/Hydraulic Sensors/Hydraulic Flow Rate
      | Sensor
  A : PMIOPort  Side=Left
  B : PMIOPort  Port=2  Side=Right
  M : PMIOPort  Port=3  Side=Right
  V : PMIOPort  Port=4  Side=Right
  connections:
  Ideal Hydraulic Flow Rate Sensor/RConn1 -- B/RConn1
  A/RConn1 -- Ideal Hydraulic Flow Rate Sensor/LConn1
  Ideal Hydraulic Flow Rate Sensor/RConn2 -- M/RConn1
  Ideal Hydraulic Flow Rate Sensor/RConn3 -- V/RConn1

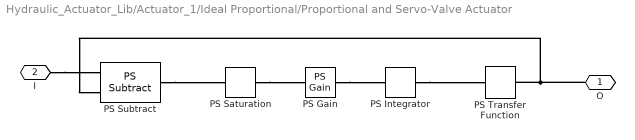
== system Hydraulic_Actuator_Lib/Actuator_1/Ideal Proportional/Proportional and Servo-Valve Actuator ==
  PS Gain : fl_lib/Physical Signals/Functions/PS Gain  gain=WT_Params.Pitch_Actuator.Servo.gain 1/s
  PS Integrator : fl_lib/Physical Signals/Linear Operators/PS Integrator  reset_method=foundation.enum.IntegratorResetSpec.None  initial_condition_spec=foundation.enum.IntegratorICSpec.Internal  saturation_spec=foundation.enum.IntegratorSaturationSpec.None  saturation_source_spec=foundation.enum.IntegratorSaturationSourceSpec.Internal  x0=0  xu=inf s  xl=-inf s
  PS Saturation : fl_lib/Physical Signals/Nonlinear Operators/PS Saturation  upper_limit=WT_Params.Pitch_Actuator.Servo.saturation  lower_limit=-(WT_Params.Pitch_Actuator.Servo.saturation)  ZeroCross=true
  PS Subtract : fl_lib/Physical Signals/Functions/PS Subtract
      settings: LibrarySourceBlock=|
      | sh_lib/Valves/Valve Actuators/Proportional and
      | Servo-Valve Actuator
  PS Transfer Function : fl_lib/Physical Signals/Linear Operators/PS Transfer Function  transfer_function_type=foundation.enum.transfer_function_type.lag  T=WT_Params.Pitch_Actuator.Servo.time_constant s  T1=2 s  T2=1 s  reset_method=foundation.enum.IntegratorResetSpec.None  initial_condition_spec=foundation.enum.IntegratorICSpec.Internal  y0=0
      settings: InternalSimscapePortConfiguration="{\"Bottom\":[],\"Left\":[{\"id\":\"U\",\"label\":\"\",\"type\":\"input\"}],\"Right\":[{\"id\":\"Y\",\"label\":\"\",\"type\":\"output\"}],\"Top\":[]}"
  O : PMIOPort  Side=Right
  I : PMIOPort  Port=2  Side=Left
  connections:
  I/RConn1 -- PS Subtract/LConn1
  PS Subtract/RConn1 -- PS Saturation/LConn1
  PS Saturation/RConn1 -- PS Gain/LConn1
  PS Gain/RConn1 -- PS Integrator/LConn1
  O/RConn1 -- PS Transfer Function/RConn1 -- PS Subtract/LConn2
  PS Integrator/RConn1 -- PS Transfer Function/LConn1

== system Hydraulic_Actuator_Lib/Actuator_1/Valve Accumulator/Logic For Nominally Open ==
  PS Gain : fl_lib/Physical Signals/Functions/PS Gain  gain=-1
  PS Subtract : fl_lib/Physical Signals/Functions/PS Subtract
  Voltage_Open : fl_lib/Physical Signals/Sources/PS Constant  constant=24
  S : PMIOPort  Side=Left
  VA : PMIOPort  Port=2  Side=Right
  connections:
  VA/RConn1 -- PS Gain/RConn1
  S/RConn1 -- PS Subtract/LConn1
  PS Subtract/RConn1 -- PS Gain/LConn1
  PS Subtract/LConn2 -- Voltage_Open/RConn1

== system Hydraulic_Actuator_Lib/Actuator_1/Valve Return/Logic For Nominally Open ==
  PS Gain : fl_lib/Physical Signals/Functions/PS Gain  gain=-1
  PS Subtract : fl_lib/Physical Signals/Functions/PS Subtract
  Voltage_Open : fl_lib/Physical Signals/Sources/PS Constant  constant=24
  S : PMIOPort  Side=Left
  VA : PMIOPort  Port=2  Side=Right
  connections:
  PS Subtract/LConn2 -- Voltage_Open/RConn1
  PS Subtract/RConn1 -- PS Gain/LConn1
  S/RConn1 -- PS Subtract/LConn1
  VA/RConn1 -- PS Gain/RConn1
